simulink model "Clarke_Park_conventions"  (R2025b)
settings: Solver=VariableStepAuto  StartTime=0.0  StopTime=10.0  MaxStep=1e-3  RelTol=1e-3
settings Model: Creator=LOQ  LastModifiedBy=LOQ

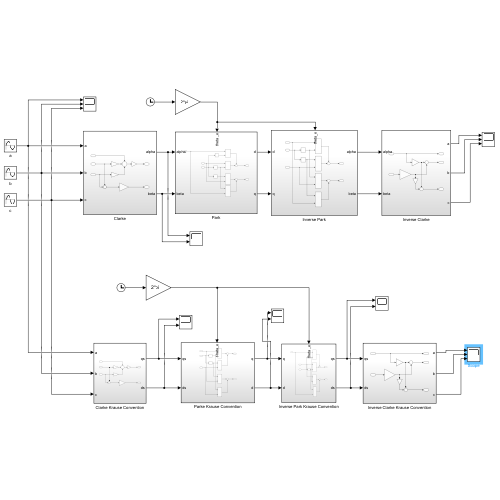
[thumbnail: Simulink's stored preview of the top-level diagram]
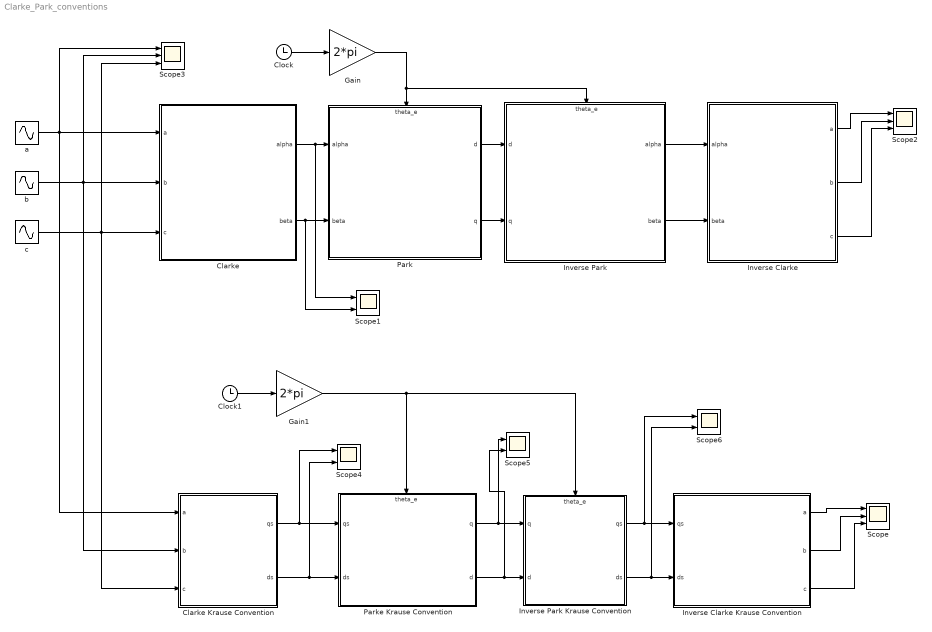
== system Clarke_Park_conventions ==
  Clarke : Subsystem
  Clarke Krause Convention : Subsystem
  Clock : Clock
  Clock1 : Clock
  Gain : Gain  Gain=2*pi
  Gain1 : Gain  Gain=2*pi
  Inverse Clarke : Subsystem
  Inverse Clarke Krause Convention : Subsystem
  Inverse Park : Subsystem
      settings: PortSchema="{\"entries\":[{\"content\":{\"sides\":[{\"content\":{\"connectorIds\":[\"In1\",\"In2\"]},\"type\":\"ConnectorPlacement.EquallySpacedRectSide\",\"uuid\":\"727c49c2-322c-4428-ae94-4dccace1ba58\"},{\"content\":{\"connectorIds\":[\"Out1\",\"Out2\"],\"side\":\"RIGHT\"},\"type\":\"ConnectorPlacement.EquallySpacedRectSide\",\"uuid\":\"a4a3860a-23f1-45ee-a3a2-be69e979ab21\"},{\"content\":{\"connectorIds\":[\"In3\"],\"side\":\"TOP\"},\"type\":\"ConnectorPlacement.EquallySpacedRectSide\",\"uuid\":\"c36ae6a8-af84-4362-94ca-46fd0807c2cb\"}]},\"type\":\"ConnectorPlacement.EquallySpacedConnector\",\"uuid\":\"3c85f25c-260c-4438-9c99-6a3b31db29b6\"}],\"packageUris\":[\"http://schema.mathworks.com/mf0/Connector/R2020b\"],\"version\":\"1.0\"}"
  Inverse Park Krause Convention : Subsystem
      settings: PortSchema="{\"entries\":[{\"content\":{\"sides\":[{\"content\":{\"connectorIds\":[\"In1\",\"In2\"]},\"type\":\"ConnectorPlacement.EquallySpacedRectSide\",\"uuid\":\"727c49c2-322c-4428-ae94-4dccace1ba58\"},{\"content\":{\"connectorIds\":[\"Out1\",\"Out2\"],\"side\":\"RIGHT\"},\"type\":\"ConnectorPlacement.EquallySpacedRectSide\",\"uuid\":\"a4a3860a-23f1-45ee-a3a2-be69e979ab21\"},{\"content\":{\"connectorIds\":[\"In3\"],\"side\":\"TOP\"},\"type\":\"ConnectorPlacement.EquallySpacedRectSide\",\"uuid\":\"c36ae6a8-af84-4362-94ca-46fd0807c2cb\"}]},\"type\":\"ConnectorPlacement.EquallySpacedConnector\",\"uuid\":\"3c85f25c-260c-4438-9c99-6a3b31db29b6\"}],\"packageUris\":[\"http://schema.mathworks.com/mf0/Connector/R2020b\"],\"version\":\"1.0\"}"
  Park : Subsystem
      settings: PortSchema="{\"entries\":[{\"content\":{\"sides\":[{\"content\":{\"connectorIds\":[\"In1\",\"In2\"]},\"type\":\"ConnectorPlacement.EquallySpacedRectSide\",\"uuid\":\"727c49c2-322c-4428-ae94-4dccace1ba58\"},{\"content\":{\"connectorIds\":[\"Out1\",\"Out2\"],\"side\":\"RIGHT\"},\"type\":\"ConnectorPlacement.EquallySpacedRectSide\",\"uuid\":\"a4a3860a-23f1-45ee-a3a2-be69e979ab21\"},{\"content\":{\"connectorIds\":[\"In3\"],\"side\":\"TOP\"},\"type\":\"ConnectorPlacement.EquallySpacedRectSide\",\"uuid\":\"c36ae6a8-af84-4362-94ca-46fd0807c2cb\"}]},\"type\":\"ConnectorPlacement.EquallySpacedConnector\",\"uuid\":\"3c85f25c-260c-4438-9c99-6a3b31db29b6\"}],\"packageUris\":[\"http://schema.mathworks.com/mf0/Connector/R2020b\"],\"version\":\"1.0\"}"
  Parke Krause Convention : Subsystem
      settings: PortSchema="{\"entries\":[{\"content\":{\"sides\":[{\"content\":{\"connectorIds\":[\"In1\",\"In2\"]},\"type\":\"ConnectorPlacement.EquallySpacedRectSide\",\"uuid\":\"727c49c2-322c-4428-ae94-4dccace1ba58\"},{\"content\":{\"connectorIds\":[\"Out1\",\"Out2\"],\"side\":\"RIGHT\"},\"type\":\"ConnectorPlacement.EquallySpacedRectSide\",\"uuid\":\"a4a3860a-23f1-45ee-a3a2-be69e979ab21\"},{\"content\":{\"connectorIds\":[\"In3\"],\"side\":\"TOP\"},\"type\":\"ConnectorPlacement.EquallySpacedRectSide\",\"uuid\":\"c36ae6a8-af84-4362-94ca-46fd0807c2cb\"}]},\"type\":\"ConnectorPlacement.EquallySpacedConnector\",\"uuid\":\"3c85f25c-260c-4438-9c99-6a3b31db29b6\"}],\"packageUris\":[\"http://schema.mathworks.com/mf0/Connector/R2020b\"],\"version\":\"1.0\"}"
  Scope : Scope  NumInputPorts=3
      settings: ActiveDisplayYMinimum=-1.2500000000000007  ActiveDisplayYMaximum=1.2500000000000031
  Scope{1,4..6} (4 alike) : Scope  NumInputPorts=2
      Scope1 settings: ActiveDisplayYMinimum=-1  ActiveDisplayYMaximum=1
      Scope4 settings: ActiveDisplayYMinimum=-1  ActiveDisplayYMaximum=1  DataLoggingVariableName=ScopeData4
      Scope5 settings: ActiveDisplayYMinimum=-1  ActiveDisplayYMaximum=1  DataLoggingVariableName=ScopeData5
      Scope6 settings: ActiveDisplayYMinimum=-1  ActiveDisplayYMaximum=1  DataLoggingVariableName=ScopeData6
  Scope2 : Scope  NumInputPorts=3
      settings: ActiveDisplayYMinimum=-7.1582044337076374  ActiveDisplayYMaximum=3.8542702214831457  DataLoggingVariableName=ScopeData2
  Scope3 : Scope  NumInputPorts=3
      settings: ActiveDisplayYMinimum=-1  ActiveDisplayYMaximum=1  DataLoggingVariableName=ScopeData3
  a : Sin  Frequency=2*pi  Phase=pi/2  SampleTime=0
  b : Sin  Frequency=2*pi  Phase=pi/2-2*pi/3  SampleTime=0
  c : Sin  Frequency=2*pi  Phase=pi/2+2*pi/3  SampleTime=0
  wires:
  a/1 -> Clarke Krause Convention/1(a), Scope3/1, Clarke/1(a)
  b/1 -> Clarke Krause Convention/2(b), Scope3/2, Clarke/2(b)
  c/1 -> Clarke Krause Convention/3(c), Scope3/3, Clarke/3(c)
  Clarke/2(beta) -> Scope1/2, Park/2(beta)
  Clarke/1(alpha) -> Scope1/1, Park/1(alpha)
  Clock/1 -> Gain/1
  Gain/1 -> Inverse Park/3(theta_e), Park/3(theta_e)
  Park/1(d) -> Inverse Park/1(d)
  Park/2(q) -> Inverse Park/2(q)
  Inverse Park/1(alpha) -> Inverse Clarke/1(alpha)
  Inverse Park/2(beta) -> Inverse Clarke/2(beta)
  Inverse Clarke/1(a) -> Scope2/1
  Inverse Clarke/2(b) -> Scope2/2
  Inverse Clarke/3(c) -> Scope2/3
  Clock1/1 -> Gain1/1
  Gain1/1 -> Inverse Park Krause Convention/3(theta_e), Parke Krause Convention/3(theta_e)
  Clarke Krause Convention/2(ds) -> Scope4/2, Parke Krause Convention/2(ds)
  Clarke Krause Convention/1(qs) -> Scope4/1, Parke Krause Convention/1(qs)
  Parke Krause Convention/1(q) -> Scope5/1, Inverse Park Krause Convention/1(q)
  Parke Krause Convention/2(d) -> Scope5/2, Inverse Park Krause Convention/2(d)
  Inverse Park Krause Convention/1(qs) -> Scope6/1, Inverse Clarke Krause Convention/1(qs)
  Inverse Park Krause Convention/2(ds) -> Scope6/2, Inverse Clarke Krause Convention/2(ds)
  Inverse Clarke Krause Convention/1(a) -> Scope/1
  Inverse Clarke Krause Convention/2(b) -> Scope/2
  Inverse Clarke Krause Convention/3(c) -> Scope/3

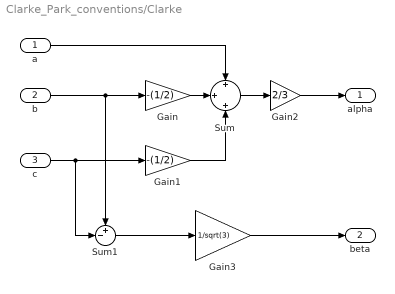
== system Clarke_Park_conventions/Clarke ==
  a : Inport
  b : Inport  Port=2
  c : Inport  Port=3
  Gain : Gain  Gain=-(1/2)
  Gain1 : Gain  Gain=-(1/2)
  Gain2 : Gain  Gain=2/3
  Gain3 : Gain  Gain=1/sqrt(3)
  Sum : Sum  Inputs=+|+|+
  Sum1 : Sum  Inputs=+-|
  alpha : Outport
  beta : Outport  Port=2
  wires:
  Gain/1 -> Sum/2
  b/1 -> Gain/1, Sum1/1
  c/1 -> Sum1/2, Gain1/1
  a/1 -> Sum/1
  Gain2/1 -> alpha/1
  Gain1/1 -> Sum/3
  Sum1/1 -> Gain3/1
  Gain3/1 -> beta/1
  Sum/1 -> Gain2/1

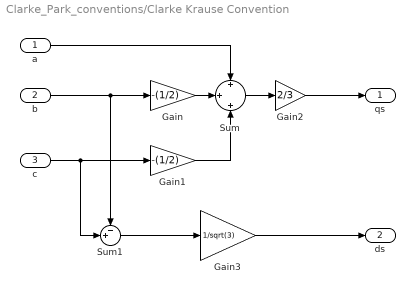
== system Clarke_Park_conventions/Clarke Krause Convention ==
  a : Inport
  b : Inport  Port=2
  c : Inport  Port=3
  Gain : Gain  Gain=-(1/2)
  Gain1 : Gain  Gain=-(1/2)
  Gain2 : Gain  Gain=2/3
  Gain3 : Gain  Gain=1/sqrt(3)
  Sum : Sum  Inputs=+|+|+
  Sum1 : Sum  Inputs=-+|
  qs : Outport
  ds : Outport  Port=2
  wires:
  b/1 -> Gain/1, Sum1/1
  Sum1/1 -> Gain3/1
  Sum/1 -> Gain2/1
  a/1 -> Sum/1
  Gain/1 -> Sum/2
  Gain3/1 -> ds/1
  Gain2/1 -> qs/1
  c/1 -> Sum1/2, Gain1/1
  Gain1/1 -> Sum/3

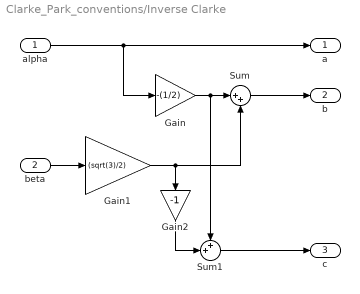
== system Clarke_Park_conventions/Inverse Clarke ==
  alpha : Inport
  beta : Inport  Port=2
  Gain : Gain  Gain=-(1/2)
  Gain1 : Gain  Gain=(sqrt(3)/2)
  Gain2 : Gain  Gain=-1
  Sum : Sum  Inputs=|++
  Sum1 : Sum  Inputs=++|
  a : Outport
  b : Outport  Port=2
  c : Outport  Port=3
  wires:
  alpha/1 -> a/1, Gain/1
  Gain2/1 -> Sum1/2
  Gain/1 -> Sum/1, Sum1/1
  Gain1/1 -> Gain2/1, Sum/2
  Sum/1 -> b/1
  beta/1 -> Gain1/1
  Sum1/1 -> c/1

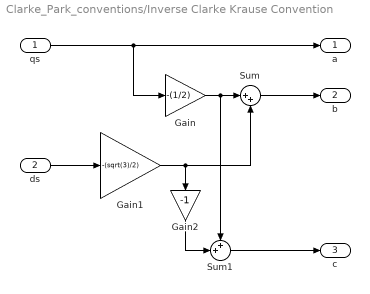
== system Clarke_Park_conventions/Inverse Clarke Krause Convention ==
  qs : Inport
  ds : Inport  Port=2
  Gain : Gain  Gain=-(1/2)
  Gain1 : Gain  Gain=-(sqrt(3)/2)
  Gain2 : Gain  Gain=-1
  Sum : Sum  Inputs=|++
  Sum1 : Sum  Inputs=++|
  a : Outport
  b : Outport  Port=2
  c : Outport  Port=3
  wires:
  qs/1 -> a/1, Gain/1
  Gain2/1 -> Sum1/2
  Gain/1 -> Sum/1, Sum1/1
  Gain1/1 -> Gain2/1, Sum/2
  Sum/1 -> b/1
  ds/1 -> Gain1/1
  Sum1/1 -> c/1

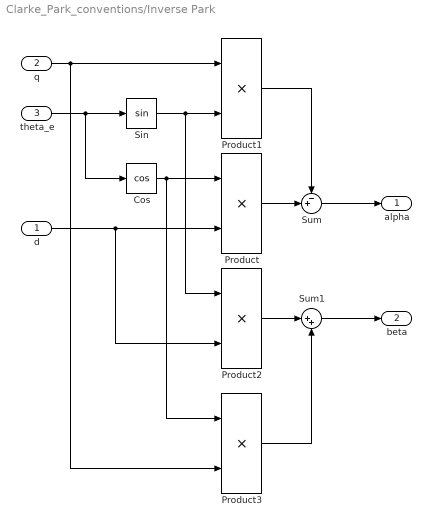
== system Clarke_Park_conventions/Inverse Park ==
  d : Inport
  q : Inport  Port=2
  theta_e : Inport  Port=3
  Cos : Trigonometry  Operator=cos
  Product{,1..3} (4 alike) : Product
  Sin : Trigonometry
  Sum : Sum  Inputs=-+|
  Sum1 : Sum  Inputs=|++
  alpha : Outport
  beta : Outport  Port=2
  wires:
  q/1 -> Product3/2, Product1/1
  d/1 -> Product2/2, Product/2
  theta_e/1 -> Cos/1, Sin/1
  Sin/1 -> Product2/1, Product1/2
  Sum/1 -> alpha/1
  Cos/1 -> Product3/1, Product/1
  Product1/1 -> Sum/1
  Product/1 -> Sum/2
  Product2/1 -> Sum1/1
  Product3/1 -> Sum1/2
  Sum1/1 -> beta/1

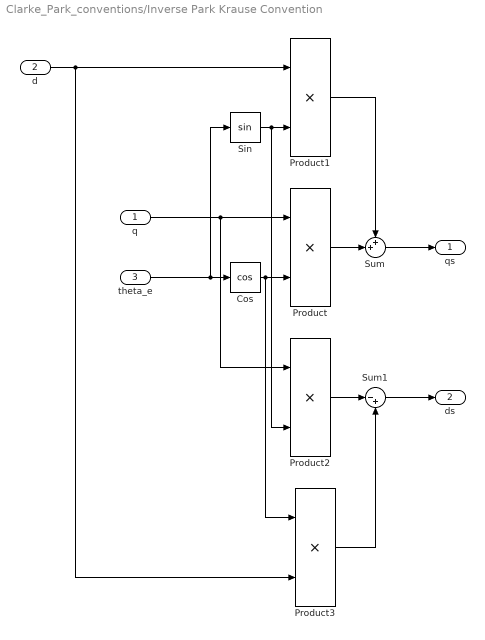
== system Clarke_Park_conventions/Inverse Park Krause Convention ==
  q : Inport
  d : Inport  Port=2
  theta_e : Inport  Port=3
  Cos : Trigonometry  Operator=cos
  Product{,1..3} (4 alike) : Product
  Sin : Trigonometry
  Sum : Sum  Inputs=++|
  Sum1 : Sum  Inputs=|-+
  qs : Outport
  ds : Outport  Port=2
  wires:
  Cos/1 -> Product3/1, Product/2
  theta_e/1 -> Sin/1, Cos/1
  q/1 -> Product2/1, Product/1
  Product1/1 -> Sum/1
  Sum/1 -> qs/1
  Product/1 -> Sum/2
  Sin/1 -> Product2/2, Product1/2
  d/1 -> Product3/2, Product1/1
  Product2/1 -> Sum1/1
  Product3/1 -> Sum1/2
  Sum1/1 -> ds/1

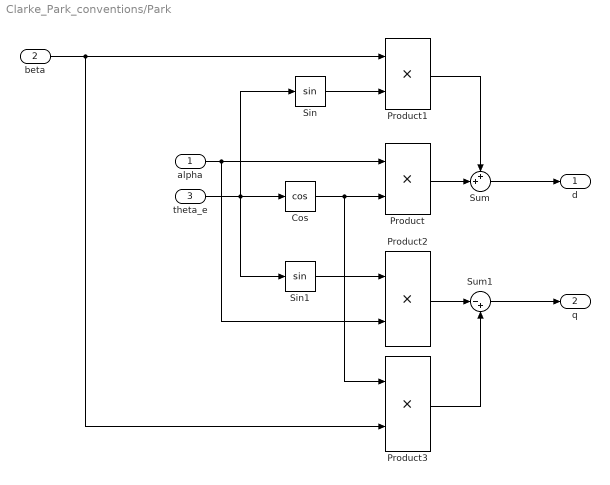
== system Clarke_Park_conventions/Park ==
  alpha : Inport
  beta : Inport  Port=2
  theta_e : Inport  Port=3
  Cos : Trigonometry  Operator=cos
  Product{,1..3} (4 alike) : Product
  Sin : Trigonometry
  Sin1 : Trigonometry
  Sum : Sum  Inputs=++|
  Sum1 : Sum  Inputs=|-+
  d : Outport
  q : Outport  Port=2
  wires:
  theta_e/1 -> Sin1/1, Sin/1, Cos/1
  Cos/1 -> Product3/1, Product/2
  Product/1 -> Sum/2
  Sin/1 -> Product1/2
  Sum/1 -> d/1
  Product1/1 -> Sum/1
  beta/1 -> Product3/2, Product1/1
  Sin1/1 -> Product2/1
  alpha/1 -> Product2/2, Product/1
  Product2/1 -> Sum1/1
  Product3/1 -> Sum1/2
  Sum1/1 -> q/1

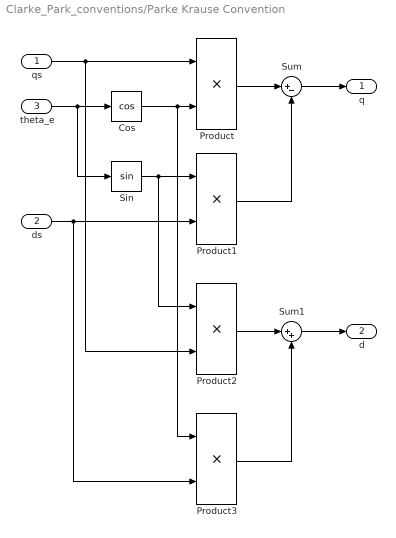
== system Clarke_Park_conventions/Parke Krause Convention ==
  qs : Inport
  ds : Inport  Port=2
  theta_e : Inport  Port=3
  Cos : Trigonometry  Operator=cos
  Product{,1..3} (4 alike) : Product
  Sin : Trigonometry
  Sum : Sum  Inputs=|+-
  Sum1 : Sum  Inputs=|++
  q : Outport
  d : Outport  Port=2
  wires:
  theta_e/1 -> Cos/1, Sin/1
  Product/1 -> Sum/1
  Product3/1 -> Sum1/2
  ds/1 -> Product3/2, Product1/2
  Cos/1 -> Product3/1, Product/2
  Product1/1 -> Sum/2
  qs/1 -> Product2/2, Product/1
  Sin/1 -> Product2/1, Product1/1
  Sum1/1 -> d/1
  Product2/1 -> Sum1/1
  Sum/1 -> q/1
